simulink model "sl_jspace"  (Simulink 7.6)
settings: Solver=ode45  StartTime=0.0  StopTime=10.0  RelTol=1e-3
libraries: roblocks x4, simulink x1
settings Model: Creator=pic  LastModifiedBy=n6334687  ExtModeTrigMode=oneshot  ExtModeArmWhenConnect=off  ExtModeAutoUpdateStatusClock=off
settings DataIOCC: LimitDataPoints=off  SignalLoggingName=sigsOut
settings OptimizationCC: BlockReduction=off  BooleanDataType=off
settings DebuggingCC: SaveWithParameterizedLinksMsg=none  SignalResolutionControl=TryResolveAllWithWarning  SolverPrmCheckMsg=none  MultiTaskDSMMsg=warning  MultiTaskCondExecSysMsg=none  StrictBusMsg=None
settings HardwareCC: TargetUnknown=on
settings RTWCC: IncludeERTFirstTime=on

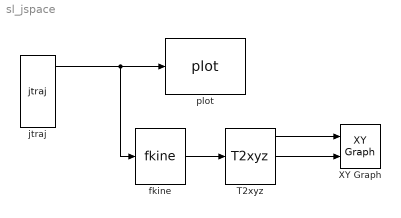
== system sl_jspace ==
  T2xyz : roblocks/Transform Conversion/T2xyz  SystemSampleTime=-1
  XY Graph : simulink/Sinks/XY Graph  SystemSampleTime=-1  xmin=-1  xmax=1  ymin=-1  ymax=1  st=-1
  fkine : roblocks/Kinematics/fkine  SystemSampleTime=-1  robot=p560
  jtraj : roblocks/Trajectory/jtraj  SystemSampleTime=-1  q0=[0 0 0 0 0 0]  qf=[pi/4 pi/2 -pi/2 0 0 0]  tmax=10
  plot : roblocks/Robot Graphics/plot  SystemSampleTime=-1  robot=p560
  wires:
  jtraj/1 -> plot/1, fkine/1
  fkine/1 -> T2xyz/1
  T2xyz/1 -> XY Graph/1
  T2xyz/2 -> XY Graph/2
